simulink model "ep2_modulator"  (R2025b)
settings: Solver=VariableStepAuto  StartTime=0.0  StopTime=10.0  RelTol=1e-3
settings Model: Creator=Fer Alexandru  LastModifiedBy=Fer Alexandru

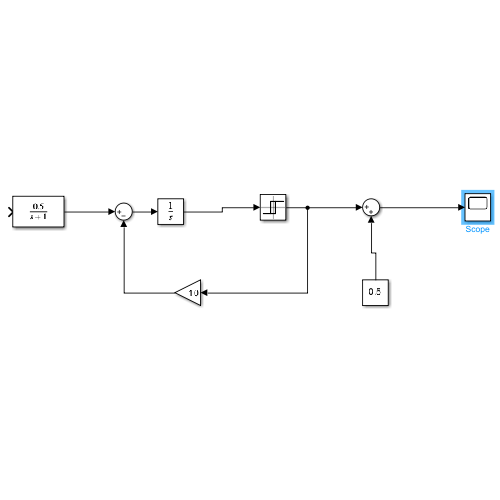
[thumbnail: Simulink's stored preview of the top-level diagram]
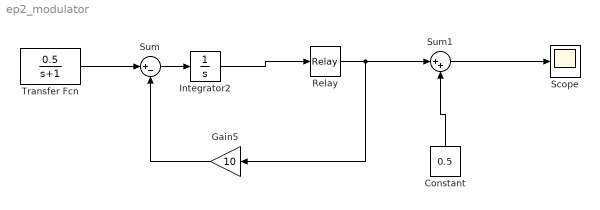
== system ep2_modulator ==
  Constant : Constant  Value=0.5
  Gain5 : Gain  Gain=10
  Integrator2 : Integrator
  Relay : Relay  OnSwitchValue=0.01  OffSwitchValue=-0.01  OnOutputValue=0.5  OffOutputValue=-0.5
  Scope : Scope
      settings: ActiveDisplayYMinimum=-0.12499999999999997  ActiveDisplayYMaximum=1.125
  Sum : Sum  Inputs=|+-
  Sum1 : Sum  Inputs=|++
  Transfer Fcn : TransferFcn  Numerator=[0.5]  Denominator=[1 1]
  wires:
  Gain5/1 -> Sum/2
  Transfer Fcn/1 -> Sum/1
  Sum/1 -> Integrator2/1
  Relay/1 -> Sum1/1, Gain5/1
  Integrator2/1 -> Relay/1
  Constant/1 -> Sum1/2
  Sum1/1 -> Scope/1
